simulink model "arducopter"  (R2021a)
settings: Solver=FixedStepAuto  StartTime=0.0  StopTime=simIn.param.timeEnd  FixedStep=simIn.param.dt  RelTol=1e-3
undefined symbols (not defined in the file or in its folder): DiscIntNeverNeededParam, sim, simIn
libraries: simulink x35, slident x4, vrlib x1
(part 6 of 9)

== system arducopter/Throttle/Throttle Calculations/Throttle-Attitude-Mixing ==
  note: This function limits the rate that thr_mix is rising with when thr_mix_des changes. It represents the function update_throttle_rpy_mix() in AC_AttitudeControl_Multi.cpp.
  note: Rate limiting of thr_mix
  note: Determination of thr_mix_des
  note: This function determines the priorization between throttle and attitude control based on the flight mode and current control demands.
      | High values favour attitude over throttle control.
      | Runs with 50 Hz.
      | ToDo: Add remaining conditions.
  thrIn : Inport
  zVelCtrlRatio : Inport  Port=2
  zVelDes : Inport  Port=3
  thrMixOut : Inport  Port=4
  thrMan : Inport  Port=5
  thrFiltIn : Inport  Port=6
  thrHover : Inport  Port=7
  Constant1 : Constant  Value=simIn.param.ATC.THR_MIX_MAX
  Constant10 : Constant  Value=1 / simIn.param.LOOP_RATE
  Constant2 : Constant  Value=simIn.param.ATC.THR_MIX_MIN
  Constant3 : Constant  Value=simIn.param.ATC.THR_MIX_MAN
  Constant4 : Constant  Value=simIn.param.ATC.THR_MIX_MAX
  Constant5 : Constant  Value=simIn.param.ATC.THR_MIX_MIN
  Data Store Memory : DataStoreMemory  DataStoreName=thrMixAct  ReadBeforeWriteMsg=warning  WriteAfterWriteMsg=warning  WriteAfterReadMsg=warning  InitialValue=simIn.init.ATC.THR_MIX  ShowAdditionalParam=off  OutDataTypeStr=single
  Update Throttle Mix : MATLAB Function  TreatAsAtomicUnit=on
  Update Throttle Mix Des : MATLAB Function  TreatAsAtomicUnit=on  SystemSampleTime=simIn.param.dt_THR_LOOP
  get_throttle_hover : Subsystem
  thrRPYMix : Outport
  wires:
  Constant1/1 -> Update Throttle Mix Des/6(thrMixMax)
  thrIn/1 -> Update Throttle Mix Des/1(thrTar)
  Update Throttle Mix Des/1(thrMixDes) -> Update Throttle Mix/1(thrMixDes)
  Constant2/1 -> Update Throttle Mix Des/5(thrMixMin)
  Constant10/1 -> Update Throttle Mix/7(dt)
  Constant3/1 -> Update Throttle Mix Des/7(thrMixMan)
  Constant5/1 -> Update Throttle Mix/2(thrMixMin)
  zVelCtrlRatio/1 -> Update Throttle Mix Des/2(zVelCtrlRatio)
  Constant4/1 -> Update Throttle Mix/3(thrMixMax)
  Update Throttle Mix/1(thrMix) -> thrRPYMix/1
  zVelDes/1 -> Update Throttle Mix Des/3(zVelDes)
  thrMan/1 -> Update Throttle Mix Des/4(thrMan)
  thrMixOut/1 -> Update Throttle Mix/4(thrOut)
  thrFiltIn/1 -> Update Throttle Mix/5(thrIn)
  thrHover/1 -> get_throttle_hover/1(in)
  get_throttle_hover/1(out) -> Update Throttle Mix/6(thrHover)

== system arducopter/Attitude Controller/input_euler_angle_roll_pitch_euler_rate_yaw()/Feedforward enabled/input shaping ==
  note: This subsystem contains all the function that are called for the input shaping of the desired attitude to calculate the target euler rates
  eulerAngleTar : Inport
  eulerInputDes : Inport  Port=2
  eulerRateTarIn : Inport  Port=3
  eulerAccelMax : Inport  Port=4
  Mux : Mux  Inputs=3
  Selector1 : Selector  InputPortWidth=3  IndexOptions=Index vector (dialog)  Indices=[1]  OutputSizes=1
  Selector2 : Selector  InputPortWidth=3  IndexOptions=Index vector (dialog)  Indices=[1]  OutputSizes=1
  Selector3 : Selector  InputPortWidth=3  IndexOptions=Index vector (dialog)  Indices=[3]  OutputSizes=1
  Selector4 : Selector  InputPortWidth=3  IndexOptions=Index vector (dialog)  Indices=[2]  OutputSizes=1
  Selector5 : Selector  InputPortWidth=3  IndexOptions=Index vector (dialog)  Indices=[2]  OutputSizes=1
  Selector6 : Selector  InputPortWidth=3  IndexOptions=Index vector (dialog)  Indices=[3]  OutputSizes=1
  Selector7 : Selector  InputPortWidth=3  IndexOptions=Index vector (dialog)  Indices=[1]  OutputSizes=1
  Selector8 : Selector  InputPortWidth=3  IndexOptions=Index vector (dialog)  Indices=[2]  OutputSizes=1
  Selector9 : Selector  InputPortWidth=3  IndexOptions=Index vector (dialog)  Indices=[3]  OutputSizes=1
  Subtract : Sum  Inputs=-+
  input shaping pitch angle : Subsystem
  input shaping roll angle : Subsystem
  input shaping yaw rate : Subsystem
  eulerRateTar : Outport
  wires:
  eulerAngleTar/1 -> Subtract/1
  eulerInputDes/1 -> Selector6/1, Subtract/2
  Subtract/1 -> Selector4/1, Selector1/1
  eulerAccelMax/1 -> Selector2/1, Selector3/1, Selector5/1
  Selector1/1 -> input shaping roll angle/1(rollAngleErr)
  Selector2/1 -> input shaping roll angle/3(rollAccelMax)
  Selector3/1 -> input shaping yaw rate/3(eulerAccelMax)
  Selector6/1 -> input shaping yaw rate/1(yawRateDes)
  eulerRateTarIn/1 -> Selector8/1, Selector9/1, Selector7/1
  Selector7/1 -> input shaping roll angle/2(rollRateTarIn)
  Selector4/1 -> input shaping pitch angle/1(pitchAngleErr)
  Selector5/1 -> input shaping pitch angle/3(pitchAccelMax)
  Selector8/1 -> input shaping pitch angle/2(pitchRateTarIn)
  Selector9/1 -> input shaping yaw rate/2(yawRateTar)
  Mux/1 -> eulerRateTar/1
  input shaping roll angle/1(eulerRollRateTar) -> Mux/1
  input shaping pitch angle/1(eulerPitchRateTar) -> Mux/2
  input shaping yaw rate/1(eulerYawRateTar) -> Mux/3

== system arducopter/Attitude Controller/input_euler_angle_roll_pitch_euler_rate_yaw()/Update attitudeTarget/Rotate target attitude ==
  attitudeTarget : Inport
  angVelTar : Inport  Port=2
  Constant : Constant  Value=simIn.param.dt
  MATLAB Function1 : MATLAB Function  TreatAsAtomicUnit=on
  MATLAB Function5 : MATLAB Function  TreatAsAtomicUnit=on
  Product : Product
  attitudeTargetRot : Outport
  wires:
  Product/1 -> MATLAB Function5/1(vec)
  angVelTar/1 -> Product/1
  Constant/1 -> Product/2
  MATLAB Function5/1(q) -> MATLAB Function1/2(q2)  "attitudeTargetUpdate"
  attitudeTarget/1 -> MATLAB Function1/1(q1)
  MATLAB Function1/1(qRes) -> attitudeTargetRot/1  "attitudeTargetRot"

== system arducopter/Attitude Controller/input_euler_angle_roll_pitch_euler_rate_yaw()/thrust_heading_rotation_angles()/Yaw error limitation ==
  note: Output adapted attitudeTarget and attitudeError if yaw limiting condition is met. Otherwise output old values.
  note: Limiting condition: if(!iszero(_p_angle_yaw.kp()) && abs(attitude_error.z) > ACCEL_Y_CONTROLLER_MAX_RADSS / _p_angle_yaw.kp())
      | --> P gain of yaw angle controller is not zero AND yaw attitude error is greater than max. yaw acceleration divided by p gain
  note: Limiting of the yaw error based on the maximum allowed yaw acceleration.
      | attitudeError and attitudeTarget are updated to include the applied limits.
  attitudeErrorIn : Inport
  thrustVecCorrection : Inport  Port=2
  attitudeBody : Inport  Port=3
  attitudeTarget : Inport  Port=4
  AND : Logic  AllPortsSameDT=off  OutDataTypeStr=boolean
  Abs : Abs
  Constant : Constant  Value=simIn.param.ATC.ACCEL_Y_CONTROLLER_MAX_RADSS
  Constant1 : Constant  Value=simIn.param.ATC.ANG_YAW_P
  Constant2 : Constant  Value=simIn.param.ATC.ANG_YAW_P
  Divide : Product  Inputs=*/
  GreaterThan : RelationalOperator  Operator=>  OutDataTypeStr=boolean  RndMeth=Simplest
  IsNonZero : simulink/Logic and Bit Operations/Compare To Zero  relop=~=  OutDataTypeStr=boolean
  Selector : Selector  InputPortWidth=3  IndexOptions=Index vector (dialog)  Indices=[3]  OutputSizes=1
  Switch : Switch  Criteria=u2 > Threshold
  Switch1 : Switch  Criteria=u2 > Threshold
  Yaw limiting and recalculation of attitudeTarget : Subsystem
  atitudeTarget : Outport
  attitudeError : Outport  Port=2
  wires:
  [attitudeError] -> Selector/1
  Constant/1 -> Divide/1
  Constant1/1 -> Divide/2
  Divide/1 -> GreaterThan/2
  Selector/1 -> Abs/1
  Abs/1 -> GreaterThan/1
  GreaterThan/1 -> AND/1
  Constant2/1 -> IsNonZero/1
  IsNonZero/1 -> AND/2
  attitudeErrorIn/1 -> [attitudeError]
  AND/1 -> Yaw limiting and recalculation of attitudeTarget/Enable, Switch1/2, Switch/2
  [attitudeError] -> Yaw limiting and recalculation of attitudeTarget/1(attitudeErrorIn)
  thrustVecCorrection/1 -> Yaw limiting and recalculation of attitudeTarget/2(thrustVecCorrection)
  attitudeBody/1 -> Yaw limiting and recalculation of attitudeTarget/3(attitudeBody)
  Yaw limiting and recalculation of attitudeTarget/1(attitudeTarget) -> Switch/1
  Yaw limiting and recalculation of attitudeTarget/2(attitudeError) -> Switch1/1
  attitudeTarget/1 -> Switch/3
  [attitudeError] -> Switch1/3
  Switch/1 -> atitudeTarget/1
  Switch1/1 -> attitudeError/1

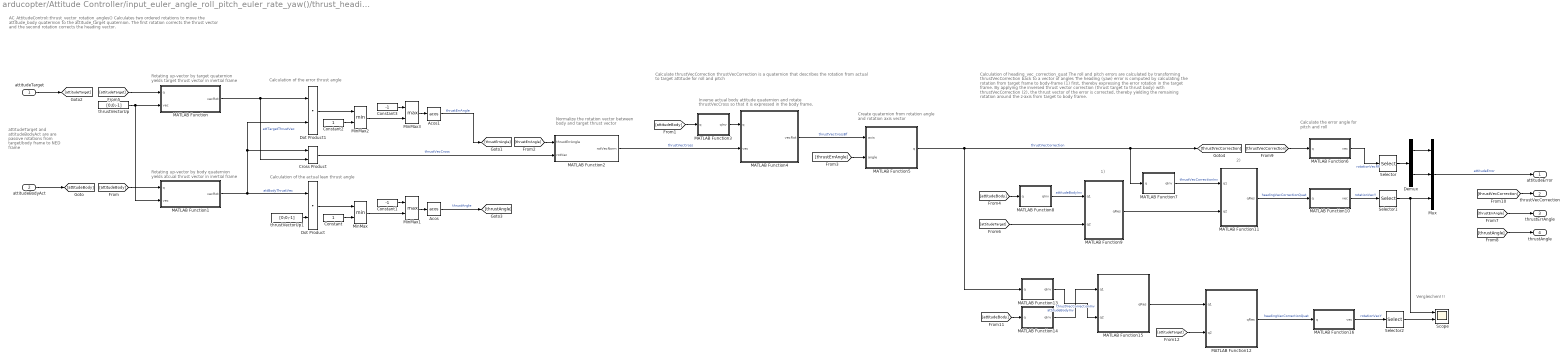
== system arducopter/Attitude Controller/input_euler_angle_roll_pitch_euler_rate_yaw()/thrust_heading_rotation_angles()/thrust_vector_rotation_angles() ==
  note: Vergleichen!!!
  note: 1)
  note: attitudeTarget and
      | attitudeBodyAct are are passive rotations from target/body frame to NED frame
  note: Calculation of heading_vec_correction_quat
      | The roll and pitch errors are calculated by transforming thrustVecCorrection back to a vector of angles
      | The heading (yaw) error is computed by calculating the rotation from target frame to body-frame (1) first, thereby expressing the error rotation in the target frame. By applying the inversed thrust vector correction (thrust target to thrust body) with thrustVecCorrection (2), the thrust vector of the error is corrected, thereby yielding the remaining rotation around the z-axis from target to body frame.
  note: Create quaternion from rotation angle and rotation axis vector
  note: Inverse actual body attitude quaternion and rotate thrustVecCross so that it is expressed in the body frame.
  note: Calculate the error angle for pitch and roll
  note: Calculate thrustVecCorrection
      | thrustVecCorrection is a quaternion that describes the rotation from actual to target attitude for roll and pitch
  note: Normalize the rotation vector between body and target thrust vector
  note: Calculation of the actual lean thrust angle
  note: Rotating up-vector by target quaternion
      | yields target thrust vector in inertial frame
  note: AC_AttitudeControl::thrust_vector_rotation_angles()
      | Calculates two ordered rotations to move the attitude_body quaternion to the attitude_target quaternion. The first rotation corrects the thrust vector and the second rotation corrects the heading vector.
  note: Rotating up-vector by body quaternion
      | yields atcual thrust vector in inertial frame
  note: Calculation of the error thrust angle
  note: 2)
  attitudeTarget : Inport
  attitudeBodyAct : Inport  Port=2
  Acos : Trigonometry  Operator=acos
  Acos1 : Trigonometry  Operator=acos
  Constant : Constant  OutDataTypeStr=single
  Constant1 : Constant  Value=-1  OutDataTypeStr=single
  Constant2 : Constant  OutDataTypeStr=single
  Constant3 : Constant  Value=-1  OutDataTypeStr=single
  Cross Product : vrlib/Utilities/Cross Product
  Demux : Demux  Outputs=2
  Dot Product : DotProduct  InputSameDT=on  OutDataTypeStr=Inherit: Inherit via internal rule
  Dot Product1 : DotProduct  InputSameDT=on  OutDataTypeStr=Inherit: Inherit via internal rule
  MATLAB Function : MATLAB Function  TreatAsAtomicUnit=on
  MATLAB Function1 : MATLAB Function  TreatAsAtomicUnit=on
  MATLAB Function10 : MATLAB Function  TreatAsAtomicUnit=on
  MATLAB Function11 : MATLAB Function  TreatAsAtomicUnit=on
  MATLAB Function12 : MATLAB Function  TreatAsAtomicUnit=on
  MATLAB Function13 : MATLAB Function  TreatAsAtomicUnit=on
  MATLAB Function14 : MATLAB Function  TreatAsAtomicUnit=on
  MATLAB Function15 : MATLAB Function  TreatAsAtomicUnit=on
  MATLAB Function16 : MATLAB Function  TreatAsAtomicUnit=on
  MATLAB Function2 : MATLAB Function  TreatAsAtomicUnit=on
  MATLAB Function3 : MATLAB Function  TreatAsAtomicUnit=on
  MATLAB Function4 : MATLAB Function  TreatAsAtomicUnit=on
  MATLAB Function5 : MATLAB Function  TreatAsAtomicUnit=on
  MATLAB Function6 : MATLAB Function  TreatAsAtomicUnit=on
  MATLAB Function7 : MATLAB Function  TreatAsAtomicUnit=on
  MATLAB Function8 : MATLAB Function  TreatAsAtomicUnit=on
  MATLAB Function9 : MATLAB Function  TreatAsAtomicUnit=on
  MinMax : MinMax  Inputs=2
  MinMax1 : MinMax  Function=max  Inputs=2
  MinMax2 : MinMax  Inputs=2
  MinMax3 : MinMax  Function=max  Inputs=2
  Mux : Mux  Inputs=3
  Scope : Scope  NumInputPorts=2
  Selector : Selector  InputPortWidth=3  IndexOptions=Index vector (dialog)  Indices=[1 2]  OutputSizes=1
  Selector1 : Selector  InputPortWidth=3  IndexOptions=Index vector (dialog)  Indices=[3]  OutputSizes=1
  Selector2 : Selector  InputPortWidth=3  IndexOptions=Index vector (dialog)  Indices=[3]  OutputSizes=1
  thrustVectorUp : Constant  Value=[0;0;-1]  OutDataTypeStr=single
  thrustVectorUp1 : Constant  Value=[0;0;-1]  OutDataTypeStr=single
  attitudeError : Outport
  thrustVecCorrection : Outport  Port=2
  thrustErrAngle : Outport  Port=3
  thrustAngle : Outport  Port=4
  wires:
  attitudeTarget/1 -> [attitudeTarget]
  thrustVectorUp/1 -> MATLAB Function1/2(vec), MATLAB Function/2(vec)
  [attitudeBody] -> MATLAB Function1/1(q)
  MATLAB Function/1(vecRot) -> Cross Product/2, Dot Product1/1  "attTargetThrustVec"
  MATLAB Function1/1(vecRot) -> Dot Product/1, Cross Product/1, Dot Product1/2  "attBodyThrustVec"
  Dot Product/1 -> MinMax/1
  MinMax/1 -> MinMax1/2
  Constant/1 -> MinMax/2
  Constant1/1 -> MinMax1/1
  MinMax1/1 -> Acos/1
  thrustVectorUp1/1 -> Dot Product/2
  Acos/1 -> [thrustAngle]  "thrustAngle"
  Constant2/1 -> MinMax2/2
  Dot Product1/1 -> MinMax2/1
  Constant3/1 -> MinMax3/1
  MinMax3/1 -> Acos1/1
  MinMax2/1 -> MinMax3/2
  Cross Product/1 -> MATLAB Function2/2(rotVec)  "thrustVecCross"
  Acos1/1 -> [thrustErrAngle]  "thrustErrAngle"
  attitudeBodyAct/1 -> [attitudeBody]
  [attitudeBody] -> MATLAB Function3/1(q)
  MATLAB Function2/1(rotVecNorm) -> MATLAB Function4/2(vec)  "thrustVecCross"
  MATLAB Function3/1(qInv) -> MATLAB Function4/1(q)
  [thrustErrAngle] -> MATLAB Function2/1(thrustErrAngle)
  MATLAB Function4/1(vecRot) -> MATLAB Function5/1(axis)  "thrustVecCrossBf"
  [thrustErrAngle] -> MATLAB Function5/2(angle)
  [attitudeBody] -> MATLAB Function8/1(q)
  [attitudeTarget] -> MATLAB Function/1(q)
  MATLAB Function7/1(qInv) -> MATLAB Function11/1(q1)  "thrustVecCorrectionInv"
  MATLAB Function8/1(qInv) -> MATLAB Function9/1(q1)  "attitudeBodyInv"
  [attitudeTarget] -> MATLAB Function9/2(q2)
  MATLAB Function11/1(qRes) -> MATLAB Function10/1(q)  "headingVecCorrectionQuat"
  MATLAB Function10/1(vec) -> Selector1/1  "rotationVecY"
  MATLAB Function6/1(vec) -> Selector/1  "rotationVecRP"
  Demux/1 -> Mux/1
  Demux/2 -> Mux/2
  Selector/1 -> Demux/1
  Selector1/1 -> Scope/1, Mux/3
  Mux/1 -> attitudeError/1  "attitudeError"
  [thrustErrAngle] -> thrustErrAngle/1
  [thrustAngle] -> thrustAngle/1
  [thrustVecCorrection] -> MATLAB Function6/1(q)
  [thrustVecCorrection] -> thrustVecCorrection/1
  [attitudeTarget] -> MATLAB Function12/2(q2)
  MATLAB Function15/1(qRes) -> MATLAB Function12/1(q1)
  MATLAB Function14/1(qInv) -> MATLAB Function15/1(q1)  "attitudeBodyInv"
  MATLAB Function13/1(qInv) -> MATLAB Function15/2(q2)  "thrustVecCorrectionInv"
  [attitudeBody] -> MATLAB Function14/1(q)
  MATLAB Function5/1(q) -> MATLAB Function13/1(q), [thrustVecCorrection], MATLAB Function7/1(q)  "thrustVecCorrection"
  MATLAB Function9/1(qRes) -> MATLAB Function11/2(q2)
  MATLAB Function12/1(qRes) -> MATLAB Function16/1(q)  "headingVecCorrectionQuat"
  MATLAB Function16/1(vec) -> Selector2/1  "rotationVecY"
  Selector2/1 -> Scope/2

== system arducopter/Attitude Controller/input_euler_angle_roll_pitch_euler_rate_yaw()/update_ang_vel_target_from_att_error()/Calc angular velocity target pitch ==
  note: Use square root controller if maximum angular acceleration is not zero
  attitudeErrorPitch : Inport
  Constant1 : Constant  Value=simIn.param.ATC.ACCEL_P_MAX
  Constant2 : Constant  Value=simIn.param.ATC.ACCEL_RP_CONTROLLER_MAX_RADSS
  Constant3 : Constant  Value=simIn.param.ATC.ACCEL_P_MAX
  Constant4 : Constant  Value=simIn.param.ATC.ACCEL_RP_CONTROLLER_MIN_RADSS
  Constant6 : Constant  Value=simIn.param.dt  VectorParams1D=off
  Constant7 : Constant  Value=simIn.param.ATC.ANG_PIT_P
  Constant8 : Constant  Value=simIn.param.ATC.ANG_PIT_P
  Gain : Gain  Gain=0.5
  Product : Product
  Saturation Dynamic : simulink/Discontinuities/Saturation Dynamic  OutMin=[]  OutMax=[]  OutDataTypeStr=Inherit: Same as second input  OutDataType=fixdt(1, 16)  OutScaling=2^-10  DoSatur=off
  Square Root Controller : MATLAB Function  TreatAsAtomicUnit=on
  Switch : Switch  Criteria=u2 > Threshold
  cdeg/ss to rad/ss1 : Gain  Gain=0.01*pi/180
  angVelPitch : Outport
  wires:
  Constant4/1 -> Saturation Dynamic/3
  Constant2/1 -> Saturation Dynamic/1
  Gain/1 -> Saturation Dynamic/2
  Constant1/1 -> Gain/1
  Saturation Dynamic/1 -> Square Root Controller/3(second_ord_lim)
  attitudeErrorPitch/1 -> Product/2, Square Root Controller/1(err)
  Product/1 -> Switch/3
  Constant6/1 -> Square Root Controller/4(dt)
  Square Root Controller/1(correction_rate) -> Switch/1
  Switch/1 -> angVelPitch/1
  Constant8/1 -> Square Root Controller/2(p)
  Constant3/1 -> cdeg/ss to rad/ss1/1
  Constant7/1 -> Product/1
  cdeg/ss to rad/ss1/1 -> Switch/2

== system arducopter/Attitude Controller/input_euler_angle_roll_pitch_euler_rate_yaw()/update_ang_vel_target_from_att_error()/Calc angular velocity target roll ==
  note: Use square root controller if maximum angular acceleration is not zero
  attitudeErrorRoll : Inport
  Constant1 : Constant  Value=simIn.param.ATC.ACCEL_R_MAX
  Constant2 : Constant  Value=simIn.param.ATC.ACCEL_RP_CONTROLLER_MAX_RADSS
  Constant3 : Constant  Value=simIn.param.ATC.ACCEL_R_MAX
  Constant4 : Constant  Value=simIn.param.ATC.ACCEL_RP_CONTROLLER_MIN_RADSS
  Constant6 : Constant  Value=simIn.param.dt  VectorParams1D=off
  Constant7 : Constant  Value=simIn.param.ATC.ANG_RLL_P
  Constant8 : Constant  Value=simIn.param.ATC.ANG_RLL_P
  Gain : Gain  Gain=0.5
  Product : Product
  Saturation Dynamic : simulink/Discontinuities/Saturation Dynamic  OutMin=[]  OutMax=[]  OutDataTypeStr=Inherit: Same as second input  OutDataType=fixdt(1, 16)  OutScaling=2^-10  DoSatur=off
  Square Root Controller : MATLAB Function  TreatAsAtomicUnit=on
  Switch : Switch  Criteria=u2 > Threshold
  cdeg/ss to rad/ss1 : Gain  Gain=0.01*pi/180
  angVelRoll : Outport
  wires:
  cdeg/ss to rad/ss1/1 -> Switch/2
  Constant7/1 -> Product/1
  Constant3/1 -> cdeg/ss to rad/ss1/1
  Constant8/1 -> Square Root Controller/2(p)
  Switch/1 -> angVelRoll/1
  Square Root Controller/1(correction_rate) -> Switch/1
  Constant6/1 -> Square Root Controller/4(dt)
  Product/1 -> Switch/3
  attitudeErrorRoll/1 -> Square Root Controller/1(err), Product/2
  Saturation Dynamic/1 -> Square Root Controller/3(second_ord_lim)
  Constant1/1 -> Gain/1
  Gain/1 -> Saturation Dynamic/2
  Constant2/1 -> Saturation Dynamic/1
  Constant4/1 -> Saturation Dynamic/3

== system arducopter/Attitude Controller/input_euler_angle_roll_pitch_euler_rate_yaw()/update_ang_vel_target_from_att_error()/Calc angular velocity target yaw ==
  note: Use square root controller if maximum angular acceleration is not zero
  attitudeErrorYaw : Inport
  Constant1 : Constant  Value=simIn.param.ATC.ACCEL_Y_MAX
  Constant2 : Constant  Value=simIn.param.ATC.ACCEL_Y_CONTROLLER_MAX_RADSS
  Constant3 : Constant  Value=simIn.param.ATC.ACCEL_Y_MAX
  Constant4 : Constant  Value=simIn.param.ATC.ACCEL_Y_CONTROLLER_MIN_RADSS
  Constant6 : Constant  Value=simIn.param.dt  VectorParams1D=off
  Constant7 : Constant  Value=simIn.param.ATC.ANG_YAW_P
  Constant8 : Constant  Value=simIn.param.ATC.ANG_YAW_P
  Gain : Gain  Gain=0.5
  Product : Product
  Saturation Dynamic : simulink/Discontinuities/Saturation Dynamic  OutMin=[]  OutMax=[]  OutDataTypeStr=Inherit: Same as second input  OutDataType=fixdt(1, 16)  OutScaling=2^-10  DoSatur=off
  Square Root Controller : MATLAB Function  TreatAsAtomicUnit=on
  Switch : Switch  Criteria=u2 > Threshold
  cdeg/ss to rad/ss1 : Gain  Gain=0.01*pi/180
  angVelYaw : Outport
  wires:
  cdeg/ss to rad/ss1/1 -> Switch/2
  Constant7/1 -> Product/1
  Constant3/1 -> cdeg/ss to rad/ss1/1
  Constant8/1 -> Square Root Controller/2(p)
  Switch/1 -> angVelYaw/1
  Square Root Controller/1(correction_rate) -> Switch/1
  Constant6/1 -> Square Root Controller/4(dt)
  Product/1 -> Switch/3
  attitudeErrorYaw/1 -> Square Root Controller/1(err), Product/2
  Saturation Dynamic/1 -> Square Root Controller/3(second_ord_lim)
  Constant1/1 -> Gain/1
  Gain/1 -> Saturation Dynamic/2
  Constant2/1 -> Saturation Dynamic/1
  Constant4/1 -> Saturation Dynamic/3

== system arducopter/Position Controller/P Position z/Set vertical speed & acceleration limit/Inverse Square Root Controller ==
  inv_sqrt_controller : TriggerPort  TriggerType=function-call  IsSimulinkFunction=on  FunctionName=inv_sqrt_controller  FunctionVisibility=scoped  VariantControl=(inherit)
  Inverse Sqrt Controller : MATLAB Function  TreatAsAtomicUnit=on
  output : ArgIn  DisableCoverage=on  OutDataTypeStr=single  ArgumentName=output
  p : ArgIn  DisableCoverage=on  Port=2  OutDataTypeStr=single  ArgumentName=p
  D_max : ArgIn  DisableCoverage=on  Port=3  OutDataTypeStr=single  ArgumentName=D_max
  err_lim : ArgOut  DisableCoverage=on  OutDataTypeStr=single  ArgumentName=err_lim
  wires:
  Inverse Sqrt Controller/1(errLim) -> err_lim/1
  output/1 -> Inverse Sqrt Controller/1(output)
  p/1 -> Inverse Sqrt Controller/2(p)
  D_max/1 -> Inverse Sqrt Controller/3(Dmax)

== system arducopter/Position Controller/PID Acceleration z/Slew Limiter/Subsystem ==
  p_out : Inport
  d_out : Inport  Port=2
  ATC sample time : Constant  Value=simIn.param.dt
  Add : Sum
  Divide : Product  Inputs=*/  OutDataTypeStr=single
  Subtract : Sum  Inputs=+-
  Unit Delay : UnitDelay  InitialCondition=simIn.init.PIDA.P + simIn.init.PIDA.D  SampleTime=-1  HasFrameUpgradeWarning=on
  sr_raw : Outport
  wires:
  ATC sample time/1 -> Divide/2
  Add/1 -> Unit Delay/1, Subtract/1
  Divide/1 -> sr_raw/1
  p_out/1 -> Add/1
  Unit Delay/1 -> Subtract/2
  Subtract/1 -> Divide/1
  d_out/1 -> Add/2

== system arducopter/Position Controller/set_pos_target_z_from_climb_rate()/input_vel_accel_z/calc accMin ==
  accMax : Inport
  Constant : Constant  Value=750  OutDataTypeStr=single
  Constant1 : Constant  Value=0  OutDataTypeStr=single
  Gain : Gain  Gain=-1
  Saturation Dynamic : simulink/Discontinuities/Saturation Dynamic  OutMin=[]  OutMax=[]  OutDataTypeStr=Inherit: Same as second input  OutDataType=fixdt(1, 16)  OutScaling=2^-10  DoSatur=off
  accMin : Outport
  wires:
  accMax/1 -> Saturation Dynamic/2
  Saturation Dynamic/1 -> Gain/1
  Gain/1 -> accMin/1
  Constant/1 -> Saturation Dynamic/1
  Constant1/1 -> Saturation Dynamic/3

== system arducopter/Position Controller/set_pos_target_z_from_climb_rate()/input_vel_accel_z/shape_vel_accel ==
  note: 1)
  note: shape_vel_accel()
      | Calculates the desired acceleration as a path from the current position, velocity and acceleration to an input velocity, considering the max velocity, acceleration and jerk.
      | Calculate KPa as time constant that defines the error decay in the kinematic path as the system approaches constant acceleration
      | Calculate the preliminary desired acceleration with the square root controller
      | Limit desired acceleration based on max. acceleration and jerk
  note: 3)
  note: 2)
  vel : Inport
  acc : Inport  Port=2
  velDes : Inport  Port=3
  accDes : Inport  Port=4
  accMin : Inport  Port=5
  accMax : Inport  Port=6
  jerkMax : Inport  Port=7
  dt : Inport  Port=8
  limitTotalAccel : Inport  Port=9
  MATLAB Function : MATLAB Function  TreatAsAtomicUnit=on
  Square Root Controller : MATLAB Function  TreatAsAtomicUnit=on
  calc_KPa : MATLAB Function  TreatAsAtomicUnit=on
  accDesShaped : Outport
  wires:
  vel/1 -> calc_KPa/1(velIn)
  acc/1 -> MATLAB Function/4(accIn)
  velDes/1 -> calc_KPa/2(vel)
  accMin/1 -> [accMin]
  accMax/1 -> [accMax]
  jerkMax/1 -> [jerkMax]
  dt/1 -> [dt]
  limitTotalAccel/1 -> MATLAB Function/8(limitTotalAccel)
  calc_KPa/2(KPa) -> Square Root Controller/2(p)
  Square Root Controller/1(correction_rate) -> MATLAB Function/1(accTar)
  MATLAB Function/1(accShaped) -> accDesShaped/1
  accDes/1 -> MATLAB Function/5(acc)
  calc_KPa/1(velErr) -> Square Root Controller/1(err)
  [dt] -> Square Root Controller/4(dt)
  [jerkMax] -> Square Root Controller/3(second_ord_lim)
  [jerkMax] -> calc_KPa/5(jerkMax)
  [dt] -> MATLAB Function/7(dt)
  [jerkMax] -> MATLAB Function/6(jerkMax)
  [accMin] -> calc_KPa/3(accMin)
  [accMax] -> calc_KPa/4(accMax)
  [accMin] -> MATLAB Function/2(accMin)
  [accMax] -> MATLAB Function/3(accMax)

== system arducopter/Position Controller/set_pos_target_z_from_climb_rate()/input_vel_accel_z/update_pos_vel_accel ==
  note: update_pos_vel_accel()
      | Single axis projection of position and velocity forwards in time based on
      | a time step of dt and acceleration off acc.
  posTarIn : Inport
  velDesIn : Inport  Port=2
  accDesIn : Inport  Port=3
  limitVectorZ : Inport  Port=4
  posErr : Inport  Port=5
  velErr : Inport  Port=6
  Constant : Constant  Value=simIn.param.dt
  MATLAB Function : MATLAB Function  TreatAsAtomicUnit=on
  posTar : Outport
  velDes : Outport  Port=2
  wires:
  posTarIn/1 -> MATLAB Function/1(posIn)
  velDesIn/1 -> MATLAB Function/2(velIn)
  accDesIn/1 -> MATLAB Function/3(accIn)
  Constant/1 -> MATLAB Function/4(dt)
  MATLAB Function/1(pos) -> posTar/1
  limitVectorZ/1 -> MATLAB Function/5(limit)
  MATLAB Function/2(vel) -> velDes/1
  posErr/1 -> MATLAB Function/6(posErr)
  velErr/1 -> MATLAB Function/7(velErr)

== system arducopter/Rate Controller/PID Pitch Rate/Slew Limiter/Subsystem ==
  p_out : Inport
  d_out : Inport  Port=2
  ATC sample time : Constant  Value=simIn.param.dt
  Add : Sum
  Divide : Product  Inputs=*/  OutDataTypeStr=single
  Subtract : Sum  Inputs=+-
  Unit Delay : UnitDelay  InitialCondition=simIn.init.PIDP.P+simIn.init.PIDP.D  SampleTime=-1  HasFrameUpgradeWarning=on
  sr_raw : Outport
  wires:
  ATC sample time/1 -> Divide/2
  Add/1 -> Unit Delay/1, Subtract/1
  Divide/1 -> sr_raw/1
  p_out/1 -> Add/1
  Unit Delay/1 -> Subtract/2
  Subtract/1 -> Divide/1
  d_out/1 -> Add/2

== system arducopter/Rate Controller/PID Roll Rate/Slew Limiter/Subsystem ==
  p_out : Inport
  d_out : Inport  Port=2
  ATC sample time : Constant  Value=simIn.param.dt
  Add : Sum
  Divide : Product  Inputs=*/  OutDataTypeStr=single
  Subtract : Sum  Inputs=+-
  Unit Delay : UnitDelay  InitialCondition=simIn.init.PIDR.P + simIn.init.PIDR.D  SampleTime=-1  HasFrameUpgradeWarning=on
  sr_raw : Outport
  wires:
  ATC sample time/1 -> Divide/2
  Add/1 -> Unit Delay/1, Subtract/1
  Divide/1 -> sr_raw/1
  p_out/1 -> Add/1
  Unit Delay/1 -> Subtract/2
  Subtract/1 -> Divide/1
  d_out/1 -> Add/2

== system arducopter/Rate Controller/PID Yaw Rate/Slew Limiter/Subsystem ==
  p_out : Inport
  d_out : Inport  Port=2
  ATC sample time : Constant  Value=simIn.param.dt
  Add : Sum
  Divide : Product  Inputs=*/  OutDataTypeStr=single
  Subtract : Sum  Inputs=+-
  Unit Delay : UnitDelay  InitialCondition=simIn.init.PIDY.P+simIn.init.PIDY.D  SampleTime=-1  HasFrameUpgradeWarning=on
  sr_raw : Outport
  wires:
  ATC sample time/1 -> Divide/2
  Add/1 -> Unit Delay/1, Subtract/1
  Divide/1 -> sr_raw/1
  p_out/1 -> Add/1
  Unit Delay/1 -> Subtract/2
  Subtract/1 -> Divide/1
  d_out/1 -> Add/2

== system arducopter/Throttle/Throttle Calculations/Throttle-Attitude-Mixing/get_throttle_hover ==
  note: get_throttle_hover()
  note: Constraining of throttle hover as executed in get_throttle_hover() (AP_MotorsMulticopter.h)
  in : Inport
  Constant : Constant  Value=simIn.param.MOT.THST_HOVER_MIN
  Constant1 : Constant  Value=simIn.param.MOT.THST_HOVER_MAX
  MATLAB Function : MATLAB Function  TreatAsAtomicUnit=on
  out : Outport
  wires:
  in/1 -> MATLAB Function/1(thrHover)
  MATLAB Function/1(thrHoverLim) -> out/1
  Constant/1 -> MATLAB Function/2(thrHoverMin)
  Constant1/1 -> MATLAB Function/3(thrHoverMax)

== system arducopter/Attitude Controller/input_euler_angle_roll_pitch_euler_rate_yaw()/Feedforward enabled/input shaping/input shaping pitch angle ==
  note: AC_AttitudeControl::input_shaping_angle(float error_angle, float input_tc, float accel_max, float target_ang_vel, float desired_ang_vel, float max_ang_vel, float dt)
      | Calculation of velocity correction from an angle error. The angular velocity has acceleration and deceleration limits including basic jerk limiting using _input_tc.
      |
      | Function is called from input_shaping_angle(float error_angle, float smoothing_gain, float accel_max, float target_ang_vel, float dt) as input_shaping_angle(error_angle, smoothing_gain, accel_max, target_ang_vel, 0.0f, 0.0f, dt), so desired_ang_vel = 0 and max_ang_vel = 0
  pitchAngleErr : Inport
  pitchRateTarIn : Inport  Port=2
  pitchAccelMax : Inport  Port=3
  Constant : Constant  Value=simIn.param.dt  VectorParams1D=off
  Constant1 : Constant  Value=simIn.param.ATC.INPUT_TC  VectorParams1D=off
  Constant2 : Constant  Value=simIn.param.dt  VectorParams1D=off
  Constant3 : Constant  Value=0  VectorParams1D=off
  Data Type Conversion : DataTypeConversion  OutDataTypeStr=single
  Data Type Conversion1 : DataTypeConversion  OutDataTypeStr=single
  MATLAB Function : MATLAB Function  TreatAsAtomicUnit=on
  MATLAB Function1 : MATLAB Function  TreatAsAtomicUnit=on
  Square Root Controller : MATLAB Function  TreatAsAtomicUnit=on
  Square Root Controller1 : Subsystem  TreatAsAtomicUnit=on
  calc p from input_tc : Subsystem
  eulerPitchRateTar : Outport
  wires:
  MATLAB Function1/1(eulerRateTar) -> eulerPitchRateTar/1
  [accelMax] -> Square Root Controller/3(second_ord_lim)
  Square Root Controller/1(correction_rate) -> MATLAB Function1/1(desiredAngVel)
  calc p from input_tc/1(p) -> Square Root Controller/2(p)
  Constant1/1 -> calc p from input_tc/1(input_tc)
  Constant/1 -> Data Type Conversion/1
  pitchAccelMax/1 -> [accelMax]
  MATLAB Function/1(radLim) -> Square Root Controller/1(err)
  pitchAngleErr/1 -> MATLAB Function/1(radIn)
  pitchRateTarIn/1 -> MATLAB Function1/2(targetAngVel)
  Data Type Conversion/1 -> Square Root Controller/4(dt)
  Data Type Conversion1/1 -> MATLAB Function1/4(dt)
  Constant2/1 -> Data Type Conversion1/1
  Constant3/1 -> MATLAB Function1/5(input_tc)
  [accelMax] -> MATLAB Function1/3(accelMax)

== system arducopter/Attitude Controller/input_euler_angle_roll_pitch_euler_rate_yaw()/Feedforward enabled/input shaping/input shaping roll angle ==
  note: AC_AttitudeControl::input_shaping_angle(float error_angle, float input_tc, float accel_max, float target_ang_vel, float desired_ang_vel, float max_ang_vel, float dt)
      | Calculation of velocity correction from an angle error. The angular velocity has acceleration and deceleration limits including basic jerk limiting using _input_tc.
      |
      | Function is called from input_shaping_angle(float error_angle, float smoothing_gain, float accel_max, float target_ang_vel, float dt) as input_shaping_angle(error_angle, smoothing_gain, accel_max, target_ang_vel, 0.0f, 0.0f, dt), so desired_ang_vel = 0 and max_ang_vel = 0
  rollAngleErr : Inport
  rollRateTarIn : Inport  Port=2
  rollAccelMax : Inport  Port=3
  Constant : Constant  Value=simIn.param.dt  VectorParams1D=off
  Constant1 : Constant  Value=simIn.param.ATC.INPUT_TC  VectorParams1D=off
  Constant2 : Constant  Value=simIn.param.dt  VectorParams1D=off
  Constant3 : Constant  Value=0  VectorParams1D=off  OutDataTypeStr=single
  Data Type Conversion : DataTypeConversion  OutDataTypeStr=single
  Data Type Conversion1 : DataTypeConversion  OutDataTypeStr=single
  MATLAB Function : MATLAB Function  TreatAsAtomicUnit=on
  MATLAB Function1 : MATLAB Function  TreatAsAtomicUnit=on
  Square Root Controller : MATLAB Function  TreatAsAtomicUnit=on
  Square Root Controller1 : Subsystem  TreatAsAtomicUnit=on
  calc p from input_tc : Subsystem
  eulerRollRateTar : Outport
  wires:
  rollAngleErr/1 -> MATLAB Function/1(radIn)
  MATLAB Function/1(radLim) -> Square Root Controller/1(err)
  rollAccelMax/1 -> [accelMax]
  Constant/1 -> Data Type Conversion/1
  Constant1/1 -> calc p from input_tc/1(input_tc)
  calc p from input_tc/1(p) -> Square Root Controller/2(p)
  Square Root Controller/1(correction_rate) -> MATLAB Function1/1(desiredAngVel)
  Constant2/1 -> Data Type Conversion1/1
  [accelMax] -> Square Root Controller/3(second_ord_lim)
  [accelMax] -> MATLAB Function1/3(accelMax)
  MATLAB Function1/1(eulerRateTar) -> eulerRollRateTar/1
  rollRateTarIn/1 -> MATLAB Function1/2(targetAngVel)
  Data Type Conversion/1 -> Square Root Controller/4(dt)
  Data Type Conversion1/1 -> MATLAB Function1/4(dt)
  Constant3/1 -> MATLAB Function1/5(input_tc)

== system arducopter/Attitude Controller/input_euler_angle_roll_pitch_euler_rate_yaw()/Feedforward enabled/input shaping/input shaping yaw rate ==
  note: AC_AttitudeControl::input_shaping_ang_vel()
      | Limits the maximum acceleration resulting from the target yaw rate, so that the target yaw rate is slewed towards the input rate
  yawRateDes : Inport
  yawRateTar : Inport  Port=2
  eulerAccelMax : Inport  Port=3
  Constant2 : Constant  Value=simIn.param.dt  VectorParams1D=off
  Constant3 : Constant  Value=simIn.param.PILOT_Y_RATE_TC  VectorParams1D=off
  Data Type Conversion1 : DataTypeConversion  OutDataTypeStr=single
  MATLAB Function1 : MATLAB Function  TreatAsAtomicUnit=on
  Square Root Controller : Subsystem  TreatAsAtomicUnit=on
  eulerYawRateTar : Outport
  wires:
  yawRateDes/1 -> MATLAB Function1/1(desiredAngVel)
  eulerAccelMax/1 -> MATLAB Function1/3(accelMax)
  MATLAB Function1/1(eulerRateTar) -> eulerYawRateTar/1
  yawRateTar/1 -> MATLAB Function1/2(targetAngVel)
  Data Type Conversion1/1 -> MATLAB Function1/4(dt)
  Constant2/1 -> Data Type Conversion1/1
  Constant3/1 -> MATLAB Function1/5(input_tc)

== system arducopter/Attitude Controller/input_euler_angle_roll_pitch_euler_rate_yaw()/thrust_heading_rotation_angles()/Yaw error limitation/Yaw limiting and recalculation of attitudeTarget ==
  note: Limit yaw error and calculate new attitudeTarget and attitudeError
  note: Create new attitudeError with limited yaw error
  note: Calculate new attitudeTarget with limited yawVecCorrection
  note: Limit yaw error based on maximum acceleration
  attitudeErrorIn : Inport
  thrustVecCorrection : Inport  Port=2
  attitudeBody : Inport  Port=3
  Enable : EnablePort
  Constant : Constant  Value=simIn.param.ATC.ACCEL_Y_CONTROLLER_MAX_RADSS
  Constant1 : Constant  Value=simIn.param.ATC.ANG_YAW_P
  Constant2 : Constant  Value=0  OutDataTypeStr=single
  Demux : Demux  Outputs=2
  Divide : Product  Inputs=*/
  Gain : Gain  Gain=-1
  MATLAB Function : MATLAB Function  TreatAsAtomicUnit=on
  MATLAB Function1 : MATLAB Function  TreatAsAtomicUnit=on
  MATLAB Function5 : MATLAB Function  TreatAsAtomicUnit=on
  MATLAB Function9 : MATLAB Function  TreatAsAtomicUnit=on
  MinMax : MinMax  Inputs=2
  MinMax1 : MinMax  Function=max  Inputs=2
  Mux : Mux  Inputs=3
  Mux1 : Mux  Inputs=3
  Selector : Selector  InputPortWidth=3  IndexOptions=Index vector (dialog)  Indices=[3]  OutputSizes=1
  Selector1 : Selector  InputPortWidth=3  IndexOptions=Index vector (dialog)  Indices=[1 2]  OutputSizes=1
  attitudeTarget : Outport
  attitudeError : Outport  Port=2
  wires:
  Constant/1 -> Divide/1
  Constant1/1 -> Divide/2
  [attitudeError] -> Selector/1
  Selector/1 -> MinMax/1
  Divide/1 -> MinMax/2, Gain/1
  MinMax/1 -> MinMax1/1
  Gain/1 -> MinMax1/2
  MinMax1/1 -> MATLAB Function/1(radIn)
  MATLAB Function/1(radLim) -> Mux1/3, Mux/3
  Constant2/1 -> Mux/2, Mux/1
  Mux/1 -> MATLAB Function5/1(vec)
  MATLAB Function5/1(q) -> MATLAB Function9/2(q2)  "yawVecCorrection"
  MATLAB Function9/1(qRes) -> MATLAB Function1/2(q2)
  thrustVecCorrection/1 -> MATLAB Function9/1(q1)
  attitudeBody/1 -> MATLAB Function1/1(q1)
  MATLAB Function1/1(qRes) -> attitudeTarget/1
  Mux1/1 -> attitudeError/1
  attitudeErrorIn/1 -> [attitudeError]
  [attitudeError] -> Selector1/1
  Selector1/1 -> Demux/1
  Demux/1 -> Mux1/1
  Demux/2 -> Mux1/2

== system arducopter/Attitude Controller/input_euler_angle_roll_pitch_euler_rate_yaw()/Feedforward enabled/input shaping/input shaping pitch angle/Square Root Controller1 ==
  sqrt_controller : TriggerPort  TriggerType=function-call  IsSimulinkFunction=on  FunctionName=sqrt_controller  FunctionVisibility=scoped  VariantControl=(inherit)
  Square Root Controller : MATLAB Function  TreatAsAtomicUnit=on
  output : ArgIn  DisableCoverage=on  OutDataTypeStr=single  ArgumentName=err
  p : ArgIn  DisableCoverage=on  Port=2  OutDataTypeStr=single  ArgumentName=p
  D_max : ArgIn  DisableCoverage=on  Port=3  OutDataTypeStr=single  ArgumentName=second_ord_lim
  output1 : ArgIn  DisableCoverage=on  Port=4  OutDataTypeStr=single  ArgumentName=dt
  correctionRate : ArgOut  DisableCoverage=on  OutDataTypeStr=single  ArgumentName=correctionRate
  wires:
  output/1 -> Square Root Controller/1(err)
  p/1 -> Square Root Controller/2(p)
  D_max/1 -> Square Root Controller/3(second_ord_lim)
  Square Root Controller/1(correction_rate) -> correctionRate/1
  output1/1 -> Square Root Controller/4(dt)

== system arducopter/Attitude Controller/input_euler_angle_roll_pitch_euler_rate_yaw()/Feedforward enabled/input shaping/input shaping pitch angle/calc p from input_tc ==
  note: Calculation of proportional factor of square root controller.
      | Based on function argument of sqrt_controller() in AC_AttitudeControl::input_shaping_angle()
  input_tc : Inport
  Constant2 : Constant  Value=0.01  OutDataTypeStr=single
  Constant3 : Constant  OutDataTypeStr=single
  Divide : Product  Inputs=*/
  Max : MinMax  Function=max  Inputs=2
  p : Outport
  wires:
  Constant2/1 -> Max/2
  Max/1 -> Divide/2
  Constant3/1 -> Divide/1
  input_tc/1 -> Max/1
  Divide/1 -> p/1

== system arducopter/Attitude Controller/input_euler_angle_roll_pitch_euler_rate_yaw()/Feedforward enabled/input shaping/input shaping roll angle/Square Root Controller1 ==
  sqrt_controller : TriggerPort  TriggerType=function-call  IsSimulinkFunction=on  FunctionName=sqrt_controller  FunctionVisibility=scoped  VariantControl=(inherit)
  Square Root Controller : MATLAB Function  TreatAsAtomicUnit=on
  output : ArgIn  DisableCoverage=on  OutDataTypeStr=single  ArgumentName=err
  p : ArgIn  DisableCoverage=on  Port=2  OutDataTypeStr=single  ArgumentName=p
  D_max : ArgIn  DisableCoverage=on  Port=3  OutDataTypeStr=single  ArgumentName=second_ord_lim
  output1 : ArgIn  DisableCoverage=on  Port=4  OutDataTypeStr=single  ArgumentName=dt
  correctionRate : ArgOut  DisableCoverage=on  OutDataTypeStr=single  ArgumentName=correctionRate
  wires:
  output/1 -> Square Root Controller/1(err)
  p/1 -> Square Root Controller/2(p)
  D_max/1 -> Square Root Controller/3(second_ord_lim)
  Square Root Controller/1(correction_rate) -> correctionRate/1
  output1/1 -> Square Root Controller/4(dt)

== system arducopter/Attitude Controller/input_euler_angle_roll_pitch_euler_rate_yaw()/Feedforward enabled/input shaping/input shaping roll angle/calc p from input_tc ==
  note: Calculation of proportional factor of square root controller.
      | Based on function argument of sqrt_controller() in AC_AttitudeControl::input_shaping_angle()
  input_tc : Inport
  Constant2 : Constant  Value=0.01  OutDataTypeStr=single
  Constant3 : Constant  OutDataTypeStr=single
  Divide : Product  Inputs=*/
  Max : MinMax  Function=max  Inputs=2
  p : Outport
  wires:
  Constant2/1 -> Max/2
  Max/1 -> Divide/2
  Constant3/1 -> Divide/1
  input_tc/1 -> Max/1
  Divide/1 -> p/1

== system arducopter/Attitude Controller/input_euler_angle_roll_pitch_euler_rate_yaw()/Feedforward enabled/input shaping/input shaping yaw rate/Square Root Controller ==
  sqrt_controller : TriggerPort  TriggerType=function-call  IsSimulinkFunction=on  FunctionName=sqrt_controller  FunctionVisibility=scoped  VariantControl=(inherit)
  Square Root Controller : MATLAB Function  TreatAsAtomicUnit=on
  output : ArgIn  DisableCoverage=on  OutDataTypeStr=single  ArgumentName=err
  p : ArgIn  DisableCoverage=on  Port=2  OutDataTypeStr=single  ArgumentName=p
  D_max : ArgIn  DisableCoverage=on  Port=3  OutDataTypeStr=single  ArgumentName=second_ord_lim
  output1 : ArgIn  DisableCoverage=on  Port=4  OutDataTypeStr=single  ArgumentName=dt
  correctionRate : ArgOut  DisableCoverage=on  OutDataTypeStr=single  ArgumentName=correctionRate
  wires:
  output/1 -> Square Root Controller/1(err)
  p/1 -> Square Root Controller/2(p)
  D_max/1 -> Square Root Controller/3(second_ord_lim)
  Square Root Controller/1(correction_rate) -> correctionRate/1
  output1/1 -> Square Root Controller/4(dt)

== matlab function arducopter/Position Controller/set_pos_target_z_from_climb_rate()/input_vel_accel_z/update_pos_vel_accel/MATLAB Function ==
  data: posIn input; pos output; velIn input; accIn input; dt input; limit input; vel output; posErr input; velErr input
function [pos, vel] = updatePosVelAccel(posIn, velIn, accIn, dt, limit, posErr, velErr)
% Single axis projection of position and velocity forwards in time based on
% a time step of dt and acceleration off acc.
% Based on update_pos_vel_accel() in control.cpp

% Move position and velocity forward by dt if it does not increase error
% when limited
pos = posIn;
deltaPos = velIn * dt + accIn * 0.5 * dt^2;
% do not add delta_pos if it will increase the velocity error in the direction of limit
if ~((deltaPos * limit) > 0 && (posErr * limit) > 0)
    pos = posIn + deltaPos;
end

% The next lines are based on update_vel_accel() which is called from
% update_pos_vel_accel()
vel = velIn;
deltaVel = accIn * dt;
% do not add delta_vel if it will increase the velocity error in the direction of limit
if ~((deltaVel * limit) > 0 && (velErr * limit) > 0)
    vel = velIn + deltaVel;
end

== matlab function arducopter/Position Controller/set z component of limit vec/MATLAB Function ==
  data: limLower input; limVecZ output; limUpper input
function limVecZ = fcn(limLower, limUpper)
% Based on AC_PosControl::update_z_controller()

if limUpper
    limVecZ = single(1);
elseif limLower
    limVecZ = single(-1);
else
    limVecZ = single(0);
end

== matlab function arducopter/Position Controller/set_pos_target_z_from_climb_rate()/input_vel_accel_z/shape_vel_accel/calc_KPa ==
  data: velErr output; velIn input; KPa output; vel input; accMin input; accMax input; jerkMax input
function [velErr, KPa] = calcKPa(velIn, vel, accMin, accMax, jerkMax)
% First part of shape_vel_accel() in control.cpp
% Calculates correction gain KPa for the square root controller based on
% the jerk and acceleration limits.

% Velocity error to be corrected
velErr = velIn - vel;

% Calculate time constants and limits to ensure stable operation.
% The direction of acceleration limit is the same as the velocity error.
% This is because the velocity error is negative when slowing down while
% closing a positive position error.
if velErr > 0
    KPa = jerkMax / accMax;
else
    KPa = jerkMax / (-accMin);
end

== matlab function arducopter/Position Controller/set_pos_target_z_from_climb_rate()/input_vel_accel_z/shape_vel_accel/Square Root Controller ==
  data: err input; correction_rate output; p input; second_ord_lim input; dt input
function correction_rate = sqrt_controller(err, p, second_ord_lim, dt)
% The square root controller
% Code is taken from sqrt_controller(...) in AC_PosControl.cpp.

if (second_ord_lim < 0 || second_ord_lim == 0)
   correction_rate = err * p;
elseif (p == 0)
    % P term is zero, but second order limit is positive
    if (err > 0)
        correction_rate = sqrt(single(2.0) * second_ord_lim * err);
    elseif (err < 0)
        correction_rate = sqrt(single(2.0) * second_ord_lim * -err);
    else
        correction_rate = single(0.0);
    end
else
    % P term and second order limit are positive, hence have been defined
    linear_dist = second_ord_lim / (p * p);
    % Check if error exceeds linear range of controller gain
    if (err > linear_dist)
        correction_rate = sqrt(single(2.0) * second_ord_lim * ( err - (linear_dist / single(2.0)) ));
    elseif (err < -linear_dist)
        correction_rate = -sqrt(single(2.0) * second_ord_lim * ( -err - (linear_dist / single(2.0)) ));
    else
        % Return linearly amplified correction if error is in linear range
        correction_rate = err * p;
    end
end

% Prevent oscillations by over-shooting the error correction in the last
% time step
if (dt ~= 0)
    correction_rate = max( min(correction_rate, abs(err) / dt), -abs(err) / dt);
end

== matlab function arducopter/Throttle/Throttle Calculations/Throttle Hover/Throttle Hover Calculation ==
  data: thrHover output single; dt input; thrAct input; zVelDes input; zVelAct input; thstHoverMax input; thstHoverMin input; thstHoverTC input; thstHoverDefault input; hoverLearn input; thrMan input; thrHoverAct data_store_memory
function thrHover = updateThrHov(dt, thrAct, zVelDes, zVelAct, thstHoverMax, thstHoverMin, thstHoverTC, thstHoverDefault, hoverLearn, thrMan)
%% Code is based on Copter::update_throttle_hover() in Attitude.cpp

global thrHoverAct;

% Use default throttle hover when throttle is set to manual
if (thrMan)
    thrHoverAct = thstHoverDefault;
end
if zVelDes > 0
    thrHoverAct = thstHoverDefault;
end

% Calc average throttle if we are in level hpver
if (thrAct > 0  && abs(zVelAct) < 60)
    %% Code is based on AP_MotorsMulticopter::update_throttle_hover(dt) in AP_MotorsMulticopter.cpp
    % Update throttle hover in dependency of the current output throttle
    if ( (hoverLearn ~= 0))
        thrHoverAct = thrHoverAct + (dt / (dt + thstHoverTC) ) * (thrAct - thrHoverAct);

        % Limit throttle hover to specified limits
        thrHoverAct = max( min( thrHoverAct, thstHoverMax), thstHoverMin);
    else % Set hover to default value if learning is disabled (AP_MotorsMulticopter.cpp)
        thrHoverAct = thstHoverDefault;
    end
end

thrHover = thrHoverAct;

== matlab function arducopter/Position Controller/set_pos_target_z_from_climb_rate()/input_vel_accel_z/shape_vel_accel/MATLAB Function ==
  data: accTar input; accShaped output; accMin input; accMax input; accIn input; acc input; jerkMax input; dt input; limitTotalAccel input
function accShaped = shapeAccelDes(accTar, accMin, accMax, accIn, acc, jerkMax, dt, limitTotalAccel)
% Second part of shape_vel_accel() in control.cpp
% Constrains desired acceleration based on acceleration limits and shapes
% kinematic path according to max jerk

%% 1) Limit desired acceleration based on acceleration limits
% Constrain correction acceleration from accMin to accMax
accTar = max(min(accTar, accMax), accMin);

% Velocity correction with input velocity
accTar = accTar + accIn;

% Constrain total acceleration from accMin to accMax
if limitTotalAccel
    accTar = max(min(accTar, accMax), accMin);
end

%% 2) Calculate required jerk limited adjustment to the current acceleration
% for the next time dt. Based on shape_accel()
accDelta = accTar - acc;
if jerkMax > 0
    accDelta = max(min(accDelta, jerkMax*dt), -jerkMax*dt);
end
accShaped = acc + accDelta;

== matlab function arducopter/Position Controller/get_pilot_speed_dn()/MATLAB Function ==
  data: dnMaxIn input; dnMax output; upMax input
function dnMax = getPilotSpeedDown(dnMaxIn, upMax)
% Get maximum vertical descending velocity. Called in ModeAltHold::init()
% in the function call for AC_PosControl::set_max_speed_accel_z()
if dnMaxIn == 0
    dnMax = abs(upMax);
else
    dnMax = abs(dnMaxIn);
end

== matlab function arducopter/Attitude Controller/input_euler_angle_roll_pitch_euler_rate_yaw()/Feedforward enabled/input shaping/input shaping pitch angle/Square Root Controller1/Square Root Controller ==
  data: err input; correction_rate output; p input; second_ord_lim input; dt input
function correction_rate = sqrt_controller(err, p, second_ord_lim, dt)
% The square root controller
% Code is taken from sqrt_controller(...) in AC_PosControl.cpp.

if (second_ord_lim < 0 || second_ord_lim == 0)
   correction_rate = err * p;
elseif (p == 0)
    % P term is zero, but second order limit is positive
    if (err > 0)
        correction_rate = sqrt(single(2.0) * second_ord_lim * err);
    elseif (err < 0)
        correction_rate = sqrt(single(2.0) * second_ord_lim * -err);
    else
        correction_rate = single(0.0);
    end
else
    % P term and second order limit are positive, hence have been defined
    linear_dist = second_ord_lim / (p * p);
    % Check if error exceeds linear range of controller gain
    if (err > linear_dist)
        correction_rate = sqrt(single(2.0) * second_ord_lim * ( err - (linear_dist / single(2.0)) ));
    elseif (err < -linear_dist)
        correction_rate = -sqrt(single(2.0) * second_ord_lim * ( -err - (linear_dist / single(2.0)) ));
    else
        % Return linearly amplified correction if error is in linear range
        correction_rate = err * p;
    end
end

% Prevent oscillations by over-shooting the error correction in the last
% time step
if (dt ~= 0)
    correction_rate = max( min(correction_rate, abs(err) / dt), -abs(err) / dt);
end
